simulink subsystem "TryController"  (R2024b)
settings: Solver=VariableStepAuto  StartTime=0.0  StopTime=10.0  RelTol=1e-3
undefined symbols (not defined in the file): actuators, controlParams, DiscIntNeverNeededParam, magnetorquer, orbit, reactionWheel, spacecraft
libraries: matrix_library x5, simulink x2, vrlib x1
settings Model: Creator=marco  LastModifiedBy=domac

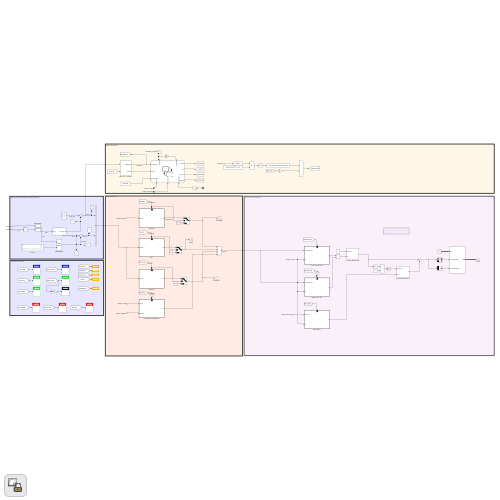
[thumbnail: Simulink's stored preview of the top-level diagram]
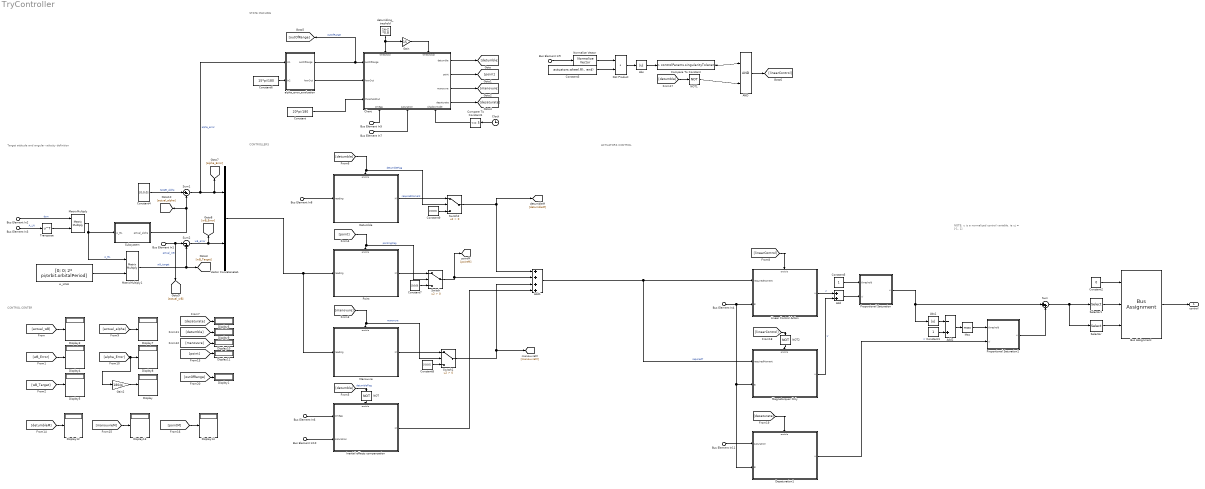
== system TryController ==
  note: STATE MACHINE
  note: ACTUATORS CONTROL
  note: CONTROLLERS
  note: CONTROL CENTER
  note: NOTE:
      | u is a normalized control variable.
      | ie uj = [-1, 1]
  note: Target attitude and angular velocity definition
  Bus Element In{1,5..6,8} (4 alike) : Inport  PortName=reading  Element=omega
  Bus Element In7 : Inport  PortName=reading  Element=saturation
  Bus Element In10 : Inport  PortName=reading  Element=saturation
  Bus Element In11 : Inport  PortName=reading  Element=saturation
  Bus Element In2 : Inport  PortName=reading  Element=dcm
  Bus Element In3 : Inport  PortName=reading  Element=lvlh
  Bus Element In4 : Inport  PortName=reading  Element=B
  Bus Element In9 : Inport  PortName=reading  Element=B
  AND : Logic  IconShape=distinctive  AllPortsSameDT=off  OutDataTypeStr=boolean
  Abs : Abs  SaturateOnIntegerOverflow=off
  Abs1 : Abs  SaturateOnIntegerOverflow=off
  Add : Sum  Inputs=2
  Add1 : Sum  Inputs=4
  Add2 : Sum  Inputs=-+
  Bus Assignment : BusAssignment  AssignedSignals=magnetorquer,reactionWheel
  Chart : Stateflow chart  TreatAsAtomicUnit=on
      settings: PortSchema="{\"entries\":[{\"content\":{\"sides\":[{\"content\":{\"connectorIds\":[\"In1\",\"In7\",\"In8\"]},\"type\":\"ConnectorPlacement.EquallySpacedRectSide\",\"uuid\":\"c6c312a3-2625-4933-bd13-ad0aab7239e3\"},{\"content\":{\"connectorIds\":[\"Out1\",\"Out2\",\"Out3\",\"Out4\"],\"side\":\"RIGHT\"},\"type\":\"ConnectorPlacement.EquallySpacedRectSide\",\"uuid\":\"85e7cf2d-51f1-4a21-b181-6f5a0be1cf34\"},{\"content\":{\"connectorIds\":[\"In5\",\"In6\"],\"side\":\"TOP\"},\"type\":\"ConnectorPlacement.EquallySpacedRectSide\",\"uuid\":\"39e679e8-5e9e-4bc0-b56b-88b23e513d0d\"},{\"content\":{\"connectorIds\":[\"In3\",\"In4\",\"In2\"],\"side\":\"BOTTOM\"},\"type\":\"ConnectorPlacement.EquallySpacedRectSide\",\"uuid\":\"37eab6da-e85c-4c6e-a698-eb2ad3d4d335\"}]},\"type\":\"ConnectorPlacement.EquallySpacedConnector\",\"uuid\":\"eda64656-7b0d-4936-ba9d-56bb47707fcc\"}],\"packageUris\":[\"http://schema.mathworks.com/mf0/Connector/R2020b\"],\"version\":\"1.0\"}"
  Clock : Clock
  Compare To Constant : simulink/Logic and Bit Operations/Compare To Constant  relop=>  const=controlParams.singularityTolerance  OutDataTypeStr=boolean
  Compare To Constant1 : simulink/Logic and Bit Operations/Compare To Constant  relop=<=  const=5  OutDataTypeStr=boolean
  Constant : Constant  Value=20*pi/180
  Constant1 : Constant
  Constant2 : Constant  Value=0  OutDataTypeStr=Bus: control
  Constant3 : Constant  Value=actuators.wheel.R(:, end)  VectorParams1D=off
  Constant4 : Constant  Value=[0;0;0]  VectorParams1D=off
  Constant5 : Constant
  Constant6 : Constant  Value=15*pi/180
  Constant7 : Constant  Value=[0;0;0]
  Constant8 : Constant  Value=[0;0;0]
  Constant9 : Constant  Value=[0;0;0]
  Desaturation1 : Subsystem
  Detumble : Subsystem
  Display{,1,3..14} (14 alike) : Display
  Dot Product : DotProduct  OutDataTypeStr=Inherit: Inherit via internal rule
  Gain : Gain  Gain=15
  Gain2 : Gain  Gain=180/pi
  Inertial effects compensation : Subsystem
  Linear Control Action : Subsystem
  "Magnetorquer Only " : Subsystem
  Manouvre : Subsystem
  MatrixMultiply : Product  Multiplication=Matrix(*)
  MatrixMultiply1 : Product  Multiplication=Matrix(*)
  Max : MinMax  Function=max
  NOT : Logic  Operator=NOT  IconShape=distinctive  AllPortsSameDT=off  OutDataTypeStr=boolean
  NOT1 : Logic  Operator=NOT  IconShape=distinctive  AllPortsSameDT=off  OutDataTypeStr=boolean
  NOT2 : Logic  Operator=NOT  IconShape=distinctive  AllPortsSameDT=off  OutDataTypeStr=boolean
  Normalize Vector : vrlib/Utilities/Normalize Vector  maxzero=0
  Point : Subsystem
  Proportional Saturation : Subsystem
  Proportional Saturation1 : Subsystem
  Selector : Selector  InputPortWidth=4  IndexOptions=Index vector (dialog)  Indices=4  OutputSizes=1
  Selector1 : Selector  InputPortWidth=4  IndexOptions=Index vector (dialog)  Indices=[1 2 3]  OutputSizes=1
  Subsystem : Subsystem
  Sum : Sum  Inputs=|++
  Sum1 : Sum  Inputs=|+-
  Sum2 : Sum  Inputs=|-+
  Switch : Switch  Criteria=u2 > Threshold  SaturateOnIntegerOverflow=off  InputSameDT=off
  Switch1 : Switch  Criteria=u2 > Threshold  SaturateOnIntegerOverflow=off  InputSameDT=off
  Switch2 : Switch  Criteria=u2 > Threshold  SaturateOnIntegerOverflow=off  InputSameDT=off
  Transpose : Math  Operator=transpose
  Vector Concatenate1 : Concatenate  Mode=Multidimensional array
  alpha_error_evaluation : Subsystem
  detumbling_treshold : Constant  Value=1e-2 *0.8
  w_LVLH : Constant  Value=[0; 0; 2* pi/orbit.orbitalPeriod]  VectorParams1D=off
  control : Outport
  wires:
  Constant2/1 -> Bus Assignment/1
  Selector1/1 -> Bus Assignment/2
  Selector/1 -> Bus Assignment/3
  Bus Assignment/1 -> control/1
  detumbling_treshold/1 -> Chart/5(threshold), Gain/1
  Chart/1(detumble) -> [detumble]
  Chart/2(point) -> [point]
  Bus Element In5/1 -> Chart/3(omega)
  Bus Element In7/1 -> Chart/4(saturation)
  Chart/4(desaturate) -> [desaturate]
  Chart/3(manouvre) -> [manovure]
  Bus Element In2/1 -> MatrixMultiply/1  "dcm"
  Transpose/1 -> MatrixMultiply/2
  Point/1(M) -> Switch/1
  [point] -> Point/Enable, Switch/2  "pointingFlag"
  Vector Concatenate1/1 -> Point/1(reading), Manouvre/1(reading)
  w_LVLH/1 -> MatrixMultiply1/2
  Constant4/1 -> Sum1/1  "target_alpha"
  MatrixMultiply1/1 -> [wB_Target], Sum2/2  "wB_target"
  Sum1/1 -> [alpha_Error], Vector Concatenate1/1, alpha_error_evaluation/1(In1)  "alpha_error"
  MatrixMultiply/1 -> MatrixMultiply1/1, Subsystem/1(A_BL)  "A_BL"
  Add1/1 -> Linear Control Action/1(requiredMoment), "Magnetorquer Only "/1(requiredMoment)  "requiredT"
  Bus Element In3/1 -> Transpose/1  "A_LN"
  Sum2/1 -> [wB_Error], Vector Concatenate1/2  "wB_error"
  Bus Element In1/1 -> [actual_wB], Sum2/1  "actual_wB"
  [detumble] -> Detumble/Enable, Switch2/2  "detumbleFlag"
  [manovure] -> Manouvre/Enable, Switch1/2  "manovure"
  [actual_wB] -> Display3/1
  [wB_Error] -> Display4/1
  [wB_Target] -> Display5/1
  [actual_alpha] -> Display7/1
  [alpha_Error] -> Display8/1, Gain2/1
  [desaturate] -> Display6/1
  [detumble] -> Display9/1
  [manovure] -> Display10/1
  [point] -> Display11/1
  [detumbleM] -> Display12/1
  [manouvreM] -> Display13/1
  [pointM] -> Display14/1
  Bus Element In8/1 -> Detumble/1(reading)
  [outOfRange] -> Display1/1
  alpha_error_evaluation/1(outOfRange) -> Chart/1(outOfRange), [outOfRange]  "outOfRange"
  Gain/1 -> Chart/6(threshold2)
  Gain2/1 -> Display/1
  alpha_error_evaluation/2(howOut) -> Chart/7(howOut)
  Constant/1 -> Chart/8(thresholdOut)
  Proportional Saturation/1(u) -> Abs1/1, Sum/1
  Linear Control Action/1(u) -> Add/1  "u'"
  Bus Element In4/1 -> Linear Control Action/2(B), "Magnetorquer Only "/2(B), Desaturation1/2(B)
  Bus Element In9/1 -> Normalize Vector/1
  Constant3/1 -> Dot Product/2
  Dot Product/1 -> Abs/1
  Normalize Vector/1 -> Dot Product/1
  Compare To Constant/1 -> AND/1
  Abs/1 -> Compare To Constant/1
  Bus Element In6/1 -> Inertial effects compensation/1(omega)
  Bus Element In10/1 -> Inertial effects compensation/2(saturation)
  [detumble] -> NOT/1  "detumbleFlag"
  NOT/1 -> Inertial effects compensation/Enable
  Inertial effects compensation/1(M) -> Add1/4
  Bus Element In11/1 -> Desaturation1/1(saturation)
  [linearControl] -> NOT2/1
  [detumble] -> NOT1/1
  NOT1/1 -> AND/2
  AND/1 -> [linearControl]
  [linearControl] -> Linear Control Action/Enable
  NOT2/1 -> "Magnetorquer Only "/Enable
  [desaturate] -> Desaturation1/Enable
  "Magnetorquer Only "/1(u) -> Add/2  "u'"
  Desaturation1/1(u) -> Proportional Saturation1/2(u')  "u'"
  Add/1 -> Proportional Saturation/2(u')
  Constant5/1 -> Proportional Saturation/1(threshold)
  Max/1 -> Proportional Saturation1/1(threshold)
  Sum/1 -> Selector1/1, Selector/1
  Add2/1 -> Max/1
  Abs1/1 -> Add2/1
  Constant1/1 -> Add2/2
  Compare To Constant1/1 -> Chart/2(shadowmode)
  Clock/1 -> Compare To Constant1/1
  Proportional Saturation1/1(u) -> Sum/2
  Switch/1 -> [pointM], Add1/2
  Constant7/1 -> Switch/3
  Constant8/1 -> Switch1/3
  Switch1/1 -> Add1/3, [manouvreM]
  Constant9/1 -> Switch2/3
  Detumble/1(M) -> Switch2/1  "requiredMoment"
  Switch2/1 -> [detumbleM], Add1/1
  Subsystem/1(actual_alpha) -> [actual_alpha], Sum1/2
  Manouvre/1(M) -> Switch1/1
  Constant6/1 -> alpha_error_evaluation/2(In2)

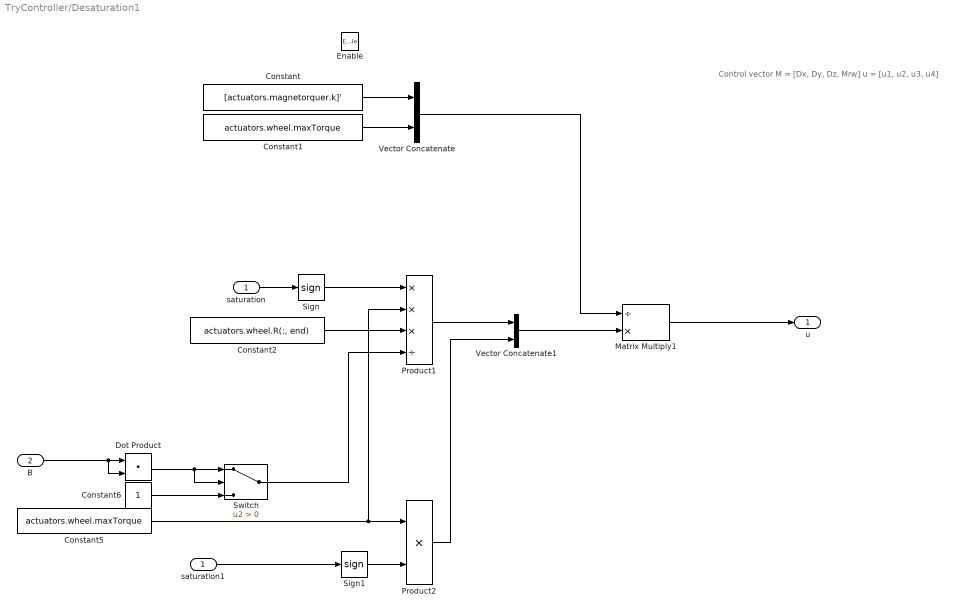
== system TryController/Desaturation1 ==
  note: Control vector
      | M = [Dx, Dy, Dz, Mrw]
      | u = [u1, u2, u3, u4]
  saturation : Inport
  B : Inport  Port=2
  Enable : EnablePort  StatesWhenEnabling=reset
  Constant : Constant  Value=[actuators.magnetorquer.k]'  VectorParams1D=off
  Constant1 : Constant  Value=actuators.wheel.maxTorque
  Constant2 : Constant  Value=actuators.wheel.R(:, end)  VectorParams1D=off
  Constant5 : Constant  Value=actuators.wheel.maxTorque
  Constant6 : Constant
  Dot Product : DotProduct  OutDataTypeStr=Inherit: Inherit via internal rule
  Matrix Multiply1 : Product  Inputs=/*
  Product1 : Product  Inputs=***/
  Product2 : Product
  Sign : Signum
  Sign1 : Signum
  Switch : Switch  Criteria=u2 > Threshold  SaturateOnIntegerOverflow=off  InputSameDT=off
  Vector Concatenate : Concatenate  Mode=Multidimensional array
  Vector Concatenate1 : Concatenate
  saturation1 : InportShadow
  u : Outport  OutMin=-1  OutMax=1  OutputWhenDisabled=reset  InitialOutput=[0;0;0;0]
  wires:
  Constant2/1 -> Product1/3
  Matrix Multiply1/1 -> u/1
  Vector Concatenate1/1 -> Matrix Multiply1/2
  Vector Concatenate/1 -> Matrix Multiply1/1
  Constant1/1 -> Vector Concatenate/2
  Constant/1 -> Vector Concatenate/1
  saturation/1 -> Sign/1
  Sign/1 -> Product1/1
  Constant5/1 -> Product2/1, Product1/2
  B/1 -> Dot Product/2, Dot Product/1
  saturation1/1 -> Sign1/1
  Sign1/1 -> Product2/2
  Product1/1 -> Vector Concatenate1/1
  Product2/1 -> Vector Concatenate1/2
  Constant6/1 -> Switch/3
  Dot Product/1 -> Switch/1, Switch/2
  Switch/1 -> Product1/4

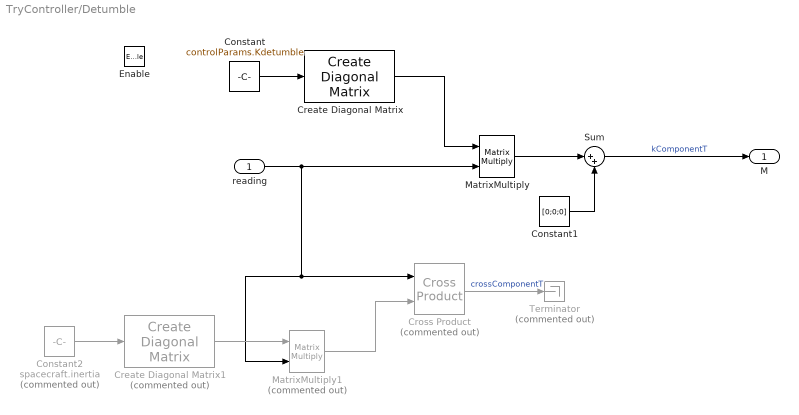
== system TryController/Detumble ==
  reading : Inport
  Enable : EnablePort  StatesWhenEnabling=reset
  Constant : Constant  Value=controlParams.Kdetumble
  Constant1 : Constant  Value=[0;0;0]
  Constant2 : Constant  Commented=on  Value=spacecraft.inertia  VectorParams1D=off
  Create Diagonal Matrix : matrix_library/Create Diagonal Matrix
  Create Diagonal Matrix1 : matrix_library/Create Diagonal Matrix  Commented=on
  Cross Product : matrix_library/Cross Product  Commented=on
  MatrixMultiply : Product  Multiplication=Matrix(*)
  MatrixMultiply1 : Product  Commented=on  Multiplication=Matrix(*)
  Sum : Sum  Inputs=|++
  Terminator : Terminator  Commented=on
  M : Outport  OutputWhenDisabled=reset  InitialOutput=[0;0;0]
  wires:
  Constant1/1 -> Sum/2
  MatrixMultiply1/1 -> Cross Product/2
  Constant/1 -> Create Diagonal Matrix/1
  Create Diagonal Matrix/1 -> MatrixMultiply/1
  Cross Product/1 -> Terminator/1  "crossComponentT"
  reading/1 -> MatrixMultiply/2, Cross Product/1, MatrixMultiply1/2
  MatrixMultiply/1 -> Sum/1
  Sum/1 -> M/1  "kComponentT"
  Create Diagonal Matrix1/1 -> MatrixMultiply1/1
  Constant2/1 -> Create Diagonal Matrix1/1

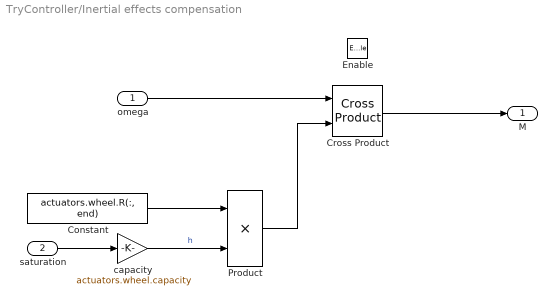
== system TryController/Inertial effects compensation ==
  omega : Inport
  saturation : Inport  Port=2
  Enable : EnablePort  StatesWhenEnabling=reset
  Constant : Constant  Value=actuators.wheel.R(:, end)  VectorParams1D=off
  Cross Product : matrix_library/Cross Product
  Product : Product
  capacity : Gain  Gain=actuators.wheel.capacity
  M : Outport  OutputWhenDisabled=reset  InitialOutput=[0;0;0]
  wires:
  Cross Product/1 -> M/1
  Product/1 -> Cross Product/2
  Constant/1 -> Product/1
  capacity/1 -> Product/2  "h"
  saturation/1 -> capacity/1
  omega/1 -> Cross Product/1

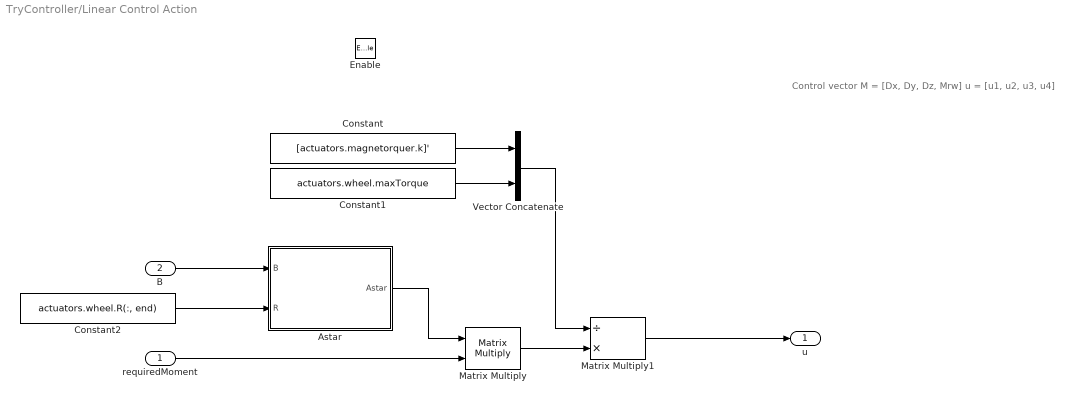
== system TryController/Linear Control Action ==
  note: Control vector
      | M = [Dx, Dy, Dz, Mrw]
      | u = [u1, u2, u3, u4]
  requiredMoment : Inport
  B : Inport  Port=2
  Enable : EnablePort  StatesWhenEnabling=reset
  Astar : Subsystem
  Constant : Constant  Value=[actuators.magnetorquer.k]'  VectorParams1D=off
  Constant1 : Constant  Value=actuators.wheel.maxTorque
  Constant2 : Constant  Value=actuators.wheel.R(:, end)  VectorParams1D=off
  Matrix Multiply : Product  Multiplication=Matrix(*)
  Matrix Multiply1 : Product  Inputs=/*
  Vector Concatenate : Concatenate  Mode=Multidimensional array
  u : Outport  OutMin=-1  OutMax=1  OutputWhenDisabled=reset  InitialOutput=[0;0;0;0]
  wires:
  Constant2/1 -> Astar/2(R)
  B/1 -> Astar/1(B)
  Matrix Multiply1/1 -> u/1
  Matrix Multiply/1 -> Matrix Multiply1/2
  Vector Concatenate/1 -> Matrix Multiply1/1
  Constant1/1 -> Vector Concatenate/2
  Constant/1 -> Vector Concatenate/1
  Astar/1(Astar) -> Matrix Multiply/1
  requiredMoment/1 -> Matrix Multiply/2

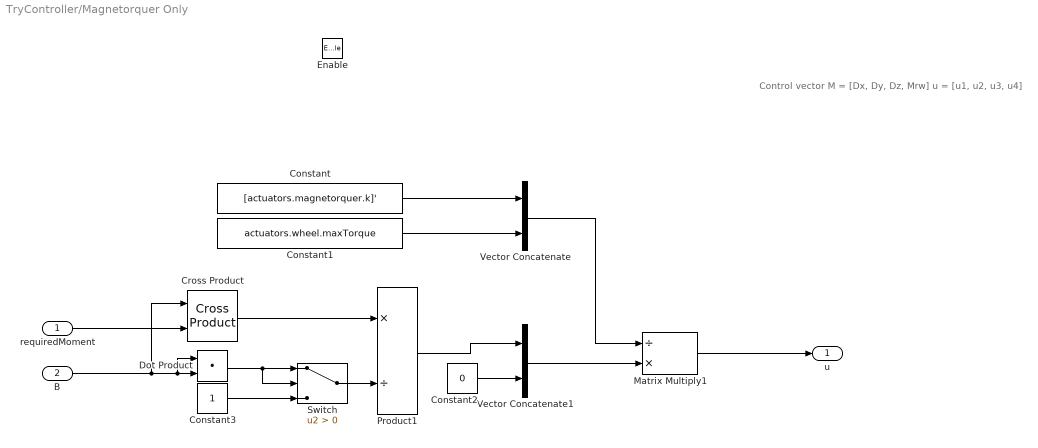
== system TryController/Magnetorquer Only  ==
  note: Control vector
      | M = [Dx, Dy, Dz, Mrw]
      | u = [u1, u2, u3, u4]
  requiredMoment : Inport
  B : Inport  Port=2
  Enable : EnablePort  StatesWhenEnabling=reset
  Constant : Constant  Value=[actuators.magnetorquer.k]'  VectorParams1D=off
  Constant1 : Constant  Value=actuators.wheel.maxTorque
  Constant2 : Constant  Value=0
  Constant3 : Constant
  Cross Product : matrix_library/Cross Product
  Dot Product : DotProduct  OutDataTypeStr=Inherit: Inherit via internal rule
  Matrix Multiply1 : Product  Inputs=/*
  Product1 : Product  Inputs=*/
  Switch : Switch  Criteria=u2 > Threshold  SaturateOnIntegerOverflow=off  InputSameDT=off
  Vector Concatenate : Concatenate  Mode=Multidimensional array
  Vector Concatenate1 : Concatenate
  u : Outport  OutMin=-1  OutMax=1  OutputWhenDisabled=reset  InitialOutput=[0;0;0;0]
  wires:
  Switch/1 -> Product1/2
  Constant3/1 -> Switch/3
  Constant2/1 -> Vector Concatenate1/2
  B/1 -> Dot Product/2, Dot Product/1, Cross Product/1
  requiredMoment/1 -> Cross Product/2
  Matrix Multiply1/1 -> u/1
  Vector Concatenate1/1 -> Matrix Multiply1/2
  Vector Concatenate/1 -> Matrix Multiply1/1
  Constant1/1 -> Vector Concatenate/2
  Constant/1 -> Vector Concatenate/1
  Cross Product/1 -> Product1/1
  Dot Product/1 -> Switch/2, Switch/1
  Product1/1 -> Vector Concatenate1/1

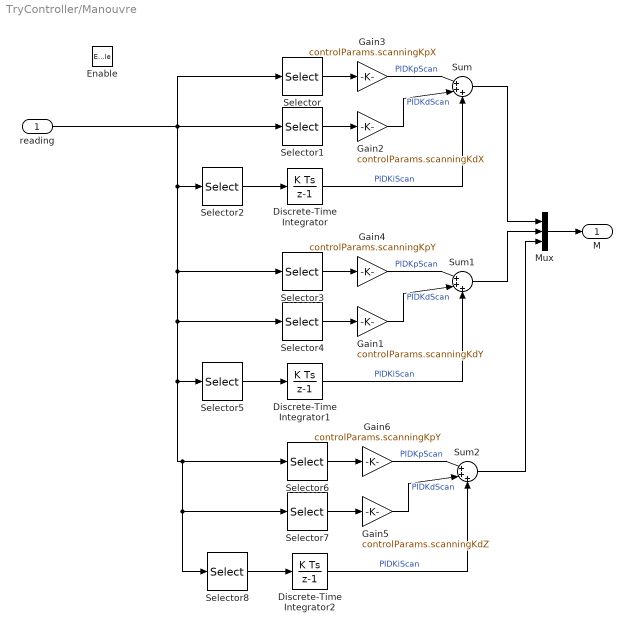
== system TryController/Manouvre ==
  reading : Inport
  Enable : EnablePort  StatesWhenEnabling=reset
  Discrete-Time Integrator : DiscreteIntegrator  gainval=controlParams.scanningKiX  SampleTime=-1  ICPrevOutput=DiscIntNeverNeededParam  ICPrevScaledInput=DiscIntNeverNeededParam
  Discrete-Time Integrator1 : DiscreteIntegrator  gainval=controlParams.scanningKiY  SampleTime=-1  ICPrevOutput=DiscIntNeverNeededParam  ICPrevScaledInput=DiscIntNeverNeededParam
  Discrete-Time Integrator2 : DiscreteIntegrator  gainval=controlParams.scanningKiZ  SampleTime=-1  ICPrevOutput=DiscIntNeverNeededParam  ICPrevScaledInput=DiscIntNeverNeededParam
  Gain1 : Gain  Gain=controlParams.scanningKdY
  Gain2 : Gain  Gain=controlParams.scanningKdX
  Gain3 : Gain  Gain=controlParams.scanningKpX
  Gain4 : Gain  Gain=controlParams.scanningKpY
  Gain5 : Gain  Gain=controlParams.scanningKdZ
  Gain6 : Gain  Gain=controlParams.scanningKpY
  Mux : Mux  Inputs=3
  Selector : Selector  InputPortWidth=6  IndexOptions=Index vector (dialog)  Indices=[1]  OutputSizes=1
  Selector1 : Selector  InputPortWidth=6  IndexOptions=Index vector (dialog)  Indices=4  OutputSizes=1
  Selector2 : Selector  InputPortWidth=6  IndexOptions=Index vector (dialog)  Indices=1  OutputSizes=1
  Selector3 : Selector  InputPortWidth=6  IndexOptions=Index vector (dialog)  Indices=2  OutputSizes=1
  Selector4 : Selector  InputPortWidth=6  IndexOptions=Index vector (dialog)  Indices=5  OutputSizes=1
  Selector5 : Selector  InputPortWidth=6  IndexOptions=Index vector (dialog)  Indices=2  OutputSizes=1
  Selector6 : Selector  InputPortWidth=6  IndexOptions=Index vector (dialog)  Indices=3  OutputSizes=1
  Selector7 : Selector  InputPortWidth=6  IndexOptions=Index vector (dialog)  Indices=6  OutputSizes=1
  Selector8 : Selector  InputPortWidth=6  IndexOptions=Index vector (dialog)  Indices=3  OutputSizes=1
  Sum : Sum  Inputs=|+++
  Sum1 : Sum  Inputs=|+++
  Sum2 : Sum  Inputs=|+++
  M : Outport
  wires:
  Sum2/1 -> Mux/3
  Sum1/1 -> Mux/2
  Sum/1 -> Mux/1
  Mux/1 -> M/1
  Gain6/1 -> Sum2/1  "PIDKpScan"
  Selector7/1 -> Gain5/1
  reading/1 -> Selector/1, Selector1/1, Selector2/1, Selector3/1, Selector6/1, Selector8/1, Selector7/1, Selector5/1, Selector4/1
  Selector6/1 -> Gain6/1
  Gain5/1 -> Sum2/2  "PIDKdScan"
  Selector8/1 -> Discrete-Time Integrator2/1
  Discrete-Time Integrator2/1 -> Sum2/3  "PIDKiScan"
  Gain4/1 -> Sum1/1  "PIDKpScan"
  Selector4/1 -> Gain1/1
  Selector3/1 -> Gain4/1
  Gain1/1 -> Sum1/2  "PIDKdScan"
  Selector5/1 -> Discrete-Time Integrator1/1
  Discrete-Time Integrator1/1 -> Sum1/3  "PIDKiScan"
  Selector2/1 -> Discrete-Time Integrator/1
  Discrete-Time Integrator/1 -> Sum/3  "PIDKiScan"
  Gain2/1 -> Sum/2  "PIDKdScan"
  Selector/1 -> Gain3/1
  Selector1/1 -> Gain2/1
  Gain3/1 -> Sum/1  "PIDKpScan"

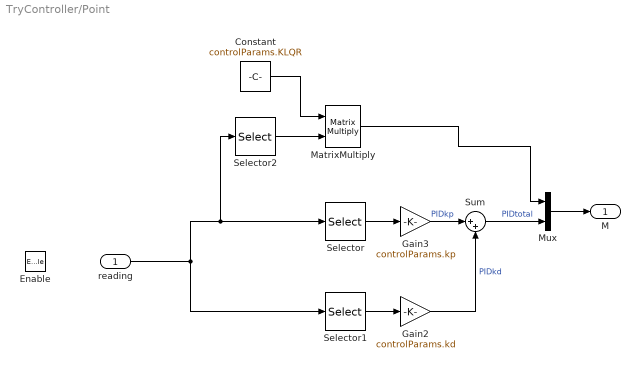
== system TryController/Point ==
  reading : Inport
  Enable : EnablePort  StatesWhenEnabling=reset
  Constant : Constant  Value=controlParams.KLQR
  Gain2 : Gain  Gain=controlParams.kd
  Gain3 : Gain  Gain=controlParams.kp
  MatrixMultiply : Product  Multiplication=Matrix(*)
  Mux : Mux  Inputs=2
  Selector : Selector  InputPortWidth=6  IndexOptions=Index vector (dialog)  Indices=[3]  OutputSizes=1
  Selector1 : Selector  InputPortWidth=6  IndexOptions=Index vector (dialog)  Indices=[6]  OutputSizes=1
  Selector2 : Selector  InputPortWidth=6  IndexOptions=Index vector (dialog)  Indices=[1 2 4 5]  OutputSizes=1
  Sum : Sum  Inputs=|++
  M : Outport  OutputWhenDisabled=reset  InitialOutput=[0;0;0]
  wires:
  Mux/1 -> M/1
  MatrixMultiply/1 -> Mux/1
  Constant/1 -> MatrixMultiply/1
  Selector2/1 -> MatrixMultiply/2
  Sum/1 -> Mux/2  "PIDtotal"
  Gain3/1 -> Sum/1  "PIDkp"
  Gain2/1 -> Sum/2  "PIDkd"
  Selector/1 -> Gain3/1
  Selector1/1 -> Gain2/1
  reading/1 -> Selector2/1, Selector/1, Selector1/1

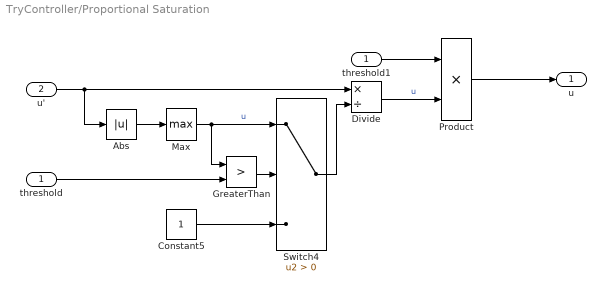
== system TryController/Proportional Saturation ==
  threshold : Inport
  u' : Inport  Port=2
  Abs : Abs  SaturateOnIntegerOverflow=off
  Constant5 : Constant
  Divide : Product  Inputs=*/
  GreaterThan : RelationalOperator  Operator=>  OutDataTypeStr=boolean  RndMeth=Simplest  InputSameDT=off
  Max : MinMax  Function=max
  Product : Product
  Switch4 : Switch  Criteria=u2 > Threshold  SaturateOnIntegerOverflow=off  InputSameDT=off
  threshold1 : InportShadow
  u : Outport
  wires:
  threshold1/1 -> Product/1
  Product/1 -> u/1
  threshold/1 -> GreaterThan/2
  Divide/1 -> Product/2  "u"
  GreaterThan/1 -> Switch4/2
  u'/1 -> Abs/1, Divide/1
  Constant5/1 -> Switch4/3
  Switch4/1 -> Divide/2
  Max/1 -> Switch4/1, GreaterThan/1  "u"
  Abs/1 -> Max/1

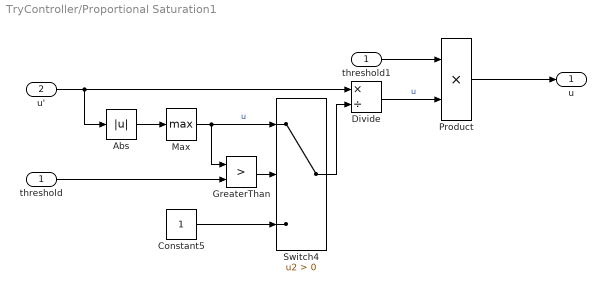
== system TryController/Proportional Saturation1 ==
  threshold : Inport
  u' : Inport  Port=2
  Abs : Abs  SaturateOnIntegerOverflow=off
  Constant5 : Constant
  Divide : Product  Inputs=*/
  GreaterThan : RelationalOperator  Operator=>  OutDataTypeStr=boolean  RndMeth=Simplest  InputSameDT=off
  Max : MinMax  Function=max
  Product : Product
  Switch4 : Switch  Criteria=u2 > Threshold  SaturateOnIntegerOverflow=off  InputSameDT=off
  threshold1 : InportShadow
  u : Outport
  wires:
  Abs/1 -> Max/1
  Max/1 -> GreaterThan/1, Switch4/1  "u"
  Switch4/1 -> Divide/2
  Constant5/1 -> Switch4/3
  u'/1 -> Divide/1, Abs/1
  GreaterThan/1 -> Switch4/2
  Divide/1 -> Product/2  "u"
  threshold/1 -> GreaterThan/2
  Product/1 -> u/1
  threshold1/1 -> Product/1

== system TryController/Subsystem ==
  A_BL : Inport
  Gain : Gain  Gain=-0.5
  Reshape : Reshape  OutputDimensionality=Column vector (2-D)
  Selector1 : Selector  InputPortWidth=9  IndexOptions=Index vector (dialog)  Indices=[6 7 2]  OutputSizes=1
  Selector2 : Selector  InputPortWidth=9  IndexOptions=Index vector (dialog)  Indices=[8 3 4]  OutputSizes=1
  Sum : Sum  Inputs=|-+
  actual_alpha : Outport
  wires:
  Sum/1 -> Gain/1  "-2a"
  Selector1/1 -> Sum/2  "-a"
  Gain/1 -> actual_alpha/1  "+a = actual_alpha"
  Reshape/1 -> Selector2/1, Selector1/1
  Selector2/1 -> Sum/1  "+a"
  A_BL/1 -> Reshape/1

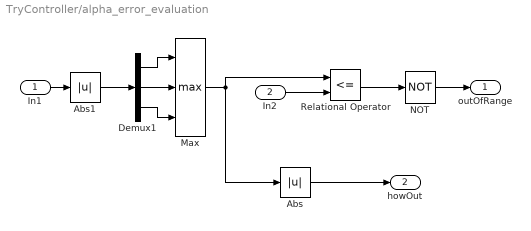
== system TryController/alpha_error_evaluation ==
  In1 : Inport
  In2 : Inport  Port=2
  Abs : Abs  SaturateOnIntegerOverflow=off
  Abs1 : Abs  SaturateOnIntegerOverflow=off
  Demux1 : Demux  Outputs=3
  Max : MinMax  Function=max  Inputs=3
  NOT : Logic  Operator=NOT  IconShape=distinctive  AllPortsSameDT=off  OutDataTypeStr=boolean
  Relational Operator : RelationalOperator  Operator=<=  OutDataTypeStr=boolean  RndMeth=Simplest  InputSameDT=off
  outOfRange : Outport
  howOut : Outport  Port=2
  wires:
  In2/1 -> Relational Operator/2
  Abs1/1 -> Demux1/1
  Abs/1 -> howOut/1
  NOT/1 -> outOfRange/1
  Relational Operator/1 -> NOT/1
  Max/1 -> Abs/1, Relational Operator/1
  Demux1/1 -> Max/1
  Demux1/3 -> Max/3
  Demux1/2 -> Max/2
  In1/1 -> Abs1/1

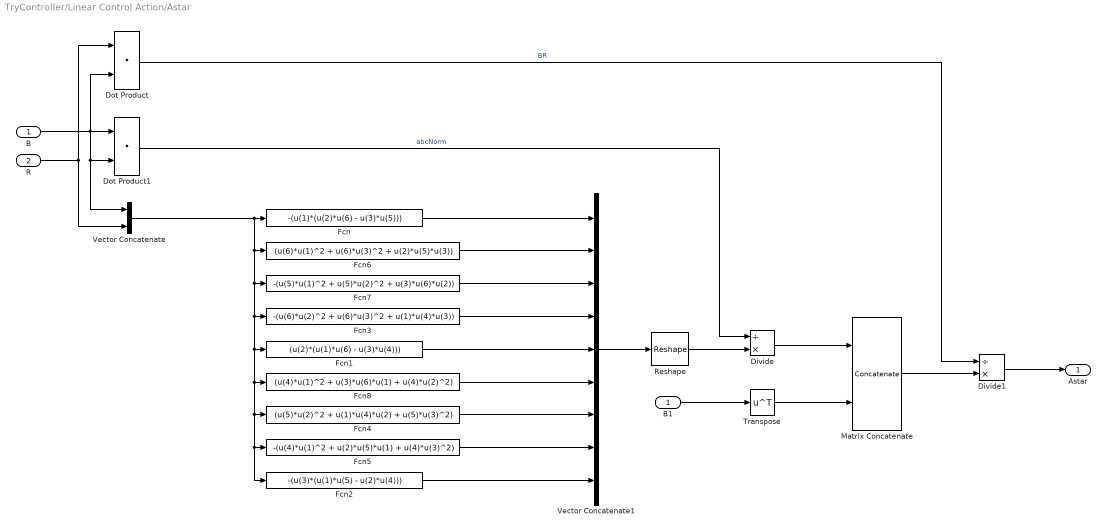
== system TryController/Linear Control Action/Astar ==
  B : Inport
  R : Inport  Port=2
  B1 : InportShadow
  Divide : Product  Inputs=/*
  Divide1 : Product  Inputs=/*
  Dot Product : DotProduct  OutDataTypeStr=Inherit: Inherit via internal rule
  Dot Product1 : DotProduct  OutDataTypeStr=Inherit: Inherit via internal rule
  Fcn : Fcn  Expr=-(u(1)*(u(2)*u(6) - u(3)*u(5)))
  Fcn1 : Fcn  Expr=(u(2)*(u(1)*u(6) - u(3)*u(4)))
  Fcn2 : Fcn  Expr=-(u(3)*(u(1)*u(5) - u(2)*u(4)))
  Fcn3 : Fcn  Expr=-(u(6)*u(2)^2 + u(6)*u(3)^2 + u(1)*u(4)*u(3))
  Fcn4 : Fcn  Expr=(u(5)*u(2)^2 + u(1)*u(4)*u(2) + u(5)*u(3)^2)
  Fcn5 : Fcn  Expr=-(u(4)*u(1)^2 + u(2)*u(5)*u(1) + u(4)*u(3)^2)
  Fcn6 : Fcn  Expr=(u(6)*u(1)^2 + u(6)*u(3)^2 + u(2)*u(5)*u(3))
  Fcn7 : Fcn  Expr=-(u(5)*u(1)^2 + u(5)*u(2)^2 + u(3)*u(6)*u(2))
  Fcn8 : Fcn  Expr=(u(4)*u(1)^2 + u(3)*u(6)*u(1) + u(4)*u(2)^2)
  Matrix Concatenate : Concatenate  Mode=Multidimensional array
  Reshape : Reshape  OutputDimensionality=Customize  OutputDimensions=[3, 3]
  Transpose : Math  Operator=transpose
  Vector Concatenate : Concatenate
  Vector Concatenate1 : Concatenate  NumInputs=9
  Astar : Outport
  wires:
  Divide1/1 -> Astar/1
  Matrix Concatenate/1 -> Divide1/2
  Transpose/1 -> Matrix Concatenate/2
  Divide/1 -> Matrix Concatenate/1
  B1/1 -> Transpose/1
  Reshape/1 -> Divide/2
  Vector Concatenate/1 -> Fcn/1, Fcn6/1, Fcn7/1, Fcn3/1, Fcn1/1, Fcn8/1, Fcn4/1, Fcn5/1, Fcn2/1
  Vector Concatenate1/1 -> Reshape/1
  Fcn2/1 -> Vector Concatenate1/9
  Fcn5/1 -> Vector Concatenate1/8
  Fcn4/1 -> Vector Concatenate1/7
  Fcn8/1 -> Vector Concatenate1/6
  Fcn1/1 -> Vector Concatenate1/5
  Fcn3/1 -> Vector Concatenate1/4
  Fcn7/1 -> Vector Concatenate1/3
  Fcn6/1 -> Vector Concatenate1/2
  Fcn/1 -> Vector Concatenate1/1
  Dot Product1/1 -> Divide/1  "abcNorm"
  Dot Product/1 -> Divide1/1  "BR"
  R/1 -> Vector Concatenate/2, Dot Product/1
  B/1 -> Dot Product1/1, Dot Product1/2, Vector Concatenate/1, Dot Product/2

== stateflow chart TryController/Chart ==
  state P2 [parallel]
    settings: executionOrder=2
    state Shadowmode
    state Detumbling
      detumble = true;
    state Detumbled
      detumble = false;
    state Manouvre
      manouvre = true;
    state Pointing
      point = true;
    (default) -> Shadowmode : {detumble = false;
        | point = false;
        | manouvre = false;
        | }
    Shadowmode -> Detumbling : [~shadowmode]
    Manouvre -> Detumbling [order 1] : [norm(omega) > threshold2]
        | {manouvre = false;}
    Detumbling -> Detumbled : [norm(omega) < threshold]
    Detumbled -> Manouvre [order 2] : [outOfRange]
        | {detumble = false;}
    Pointing -> Manouvre : [outOfRange && howOut > thresholdOut]
        | {point = false;}
    Detumbled -> Pointing [order 1] : [~outOfRange]
        | {detumble = false;}
    Manouvre -> Pointing [order 2] : [~outOfRange && norm(omega) < threshold]
        | {manouvre = false;}
  state P1 [parallel]
    settings: executionOrder=1
    state Normal
      desaturate = false;
    state Desaturation
      desaturate = true;
    (default) -> Normal
    Normal -> Desaturation : [abs(saturation) > 0.9]
    Desaturation -> Normal : [abs(saturation) < 0.2]
  data: outOfRange input; shadowmode input; detumble output; point output; manouvre output; omega input; saturation input; threshold input; desaturate output; threshold2 input; howOut input; thresholdOut input
